simulink model "Exercise_1"  (R2026a)
settings: Solver=VariableStepAuto
settings Model: Creator=thienan  LastModifiedBy=thienan

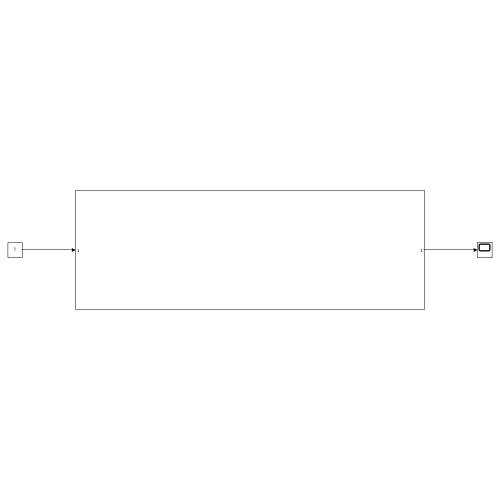
[thumbnail: Simulink's stored preview of the top-level diagram]
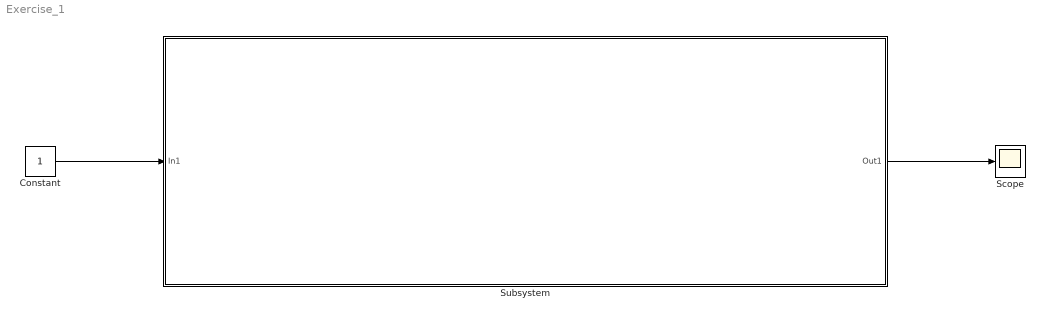
== system Exercise_1 ==
  Constant : Constant  SampleTime=0.1
  Scope : Scope
      settings: ActiveDisplayYMinimum=3.9026272650987939  ActiveDisplayYMaximum=4.0391437850073695
  Subsystem : Subsystem
  wires:
  Constant/1 -> Subsystem/1(In1)
  Subsystem/1(Out1) -> Scope/1

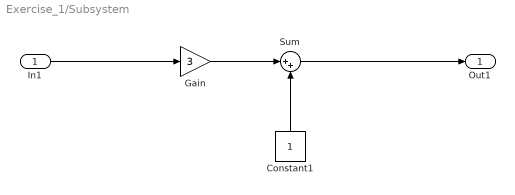
== system Exercise_1/Subsystem ==
  In1 : Inport
  Constant1 : Constant
  Gain : Gain  Gain=3
  Sum : Sum  Inputs=|++
  Out1 : Outport
  wires:
  Gain/1 -> Sum/1
  Constant1/1 -> Sum/2
  In1/1 -> Gain/1
  Sum/1 -> Out1/1
